simulink model "sf_battery_management"  (R2025b)
settings: Solver=FixedStepAuto  StartTime=0.0  StopTime=inf  FixedStep=0.1  RelTol=1e-3
PreLoadFcn:
  | load('battery_management_data.mat')
values from neighbouring files (symbols this model uses):
  CODEGEN_FLAG = 0    [battery_management_data.mat]
  currentFaultSim = 0    [battery_management_data.mat]
  currentSensorSim = 0    [battery_management_data.mat]
  tempFaultSim = 0    [battery_management_data.mat]
  tempSensorSim = 0    [battery_management_data.mat]
  voltageFaultSim = 0    [battery_management_data.mat]
  voltageSensorSim = 0    [battery_management_data.mat]
(part 3 of 3)

== stateflow chart sf_battery_management/Sensor Readings with Fault Detection ==
  state VoltageSensor [parallel]
    settings: executionOrder=1
    state SensorFaultDetection
      du: sensorError = isError(voltageRead);
      state Valid
        voltage = voltageRead;
        previousReading = voltage;
      state FaultDetected
        voltage = previousReading;
        sensorFaultDetected = true;
      state StandBy
        voltage = previousReading;
      (default) -> VoltageSensor.SensorFaultDetection.Valid
      (junction 159) -> VoltageSensor.SensorFaultDetection.Valid
      VoltageSensor.SensorFaultDetection.FaultDetected -> (junction 159) : [duration(~sensorError) > TIMEOUT]
          | {sensorFaultDetected = false;}
      VoltageSensor.SensorFaultDetection.StandBy -> VoltageSensor.SensorFaultDetection.Valid [order 1] : [~sensorError]
      VoltageSensor.SensorFaultDetection.Valid -> VoltageSensor.SensorFaultDetection.StandBy : [sensorError]
      VoltageSensor.SensorFaultDetection.StandBy -> VoltageSensor.SensorFaultDetection.FaultDetected [order 2] : [duration(sensorError) > TIMEOUT]
    VoltageSensor -> (junction 27)
    (junction 27) -> (junction 29) [order 1] : [CODEGEN_FLAG]
    (junction 27) -> (junction 94) [order 2] : %Sim behavior (dashboard blocks)
    (junction 29) -> (junction 31) : %Codegen behavior (call hardware driver C code)
        | {voltageRead = double(readVoltage())
        | voltageRead = voltageRead / 1000;}
    (junction 94) -> (junction 98) [order 1] : [voltageFaultSim >0]
    (junction 94) -> (junction 71) [order 2] : {voltageRead = voltageSensorSim;
        | voltageRead = voltageRead+VOLTAGE_NOISE*rand();}
    (junction 98) -> (junction 99) : {voltageRead = ERROR;}
    (junction 71) -> (junction 99)
    (junction 99) -> (junction 31)
  state CurrentSensor [parallel]
    settings: executionOrder=2
    state SensorFaultDetection
      du: sensorError = isError(currentRead);
      state Valid
        current = currentRead;
        previousReading = current;
      state FaultDetected
        current = previousReading;
        sensorFaultDetected = true;
      state StandBy
        current = previousReading;
      (default) -> CurrentSensor.SensorFaultDetection.Valid
      (junction 215) -> CurrentSensor.SensorFaultDetection.Valid
      CurrentSensor.SensorFaultDetection.FaultDetected -> (junction 215) : [duration(~sensorError) > TIMEOUT]
          | {sensorFaultDetected = false;}
      CurrentSensor.SensorFaultDetection.StandBy -> CurrentSensor.SensorFaultDetection.Valid [order 1] : [~sensorError]
      CurrentSensor.SensorFaultDetection.Valid -> CurrentSensor.SensorFaultDetection.StandBy : [sensorError]
      CurrentSensor.SensorFaultDetection.StandBy -> CurrentSensor.SensorFaultDetection.FaultDetected [order 2] : [duration(sensorError) > TIMEOUT]
    CurrentSensor -> (junction 111)
    (junction 111) -> (junction 110) [order 1] : [CODEGEN_FLAG]
    (junction 111) -> (junction 115) [order 2] : %Sim behavior (dashboard blocks)
    (junction 110) -> (junction 112) : %Codegen  behavior (call hardware driver C code)
        | {currentRead = double(readCurrent());
        |  currentRead = currentRead / 1000;}
    (junction 115) -> (junction 236) [order 1] : [currentFaultSim >0]
    (junction 115) -> (junction 114) [order 2] : {currentRead = currentSensorSim;
        | currentRead = currentRead+CURRENT_NOISE*rand();}
    (junction 236) -> (junction 118) : {currentRead = ERROR;}
    (junction 114) -> (junction 118)
    (junction 118) -> (junction 112)
  state TemperatureSensor [parallel]
    settings: executionOrder=3
    state SensorFaultDetection
      du: sensorError = isError(tempRead);
      state Valid
        temperature = tempRead;
        previousReading = temperature;
      state FaultDetected
        temperature = previousReading;
        sensorFaultDetected = true;
      state StandBy
        temperature = previousReading;
      (default) -> TemperatureSensor.SensorFaultDetection.Valid
      (junction 227) -> TemperatureSensor.SensorFaultDetection.Valid
      TemperatureSensor.SensorFaultDetection.FaultDetected -> (junction 227) : [duration(~sensorError) > TIMEOUT]
          | {sensorFaultDetected = false;}
      TemperatureSensor.SensorFaultDetection.StandBy -> TemperatureSensor.SensorFaultDetection.Valid [order 1] : [~sensorError]
      TemperatureSensor.SensorFaultDetection.Valid -> TemperatureSensor.SensorFaultDetection.StandBy : [sensorError]
      TemperatureSensor.SensorFaultDetection.StandBy -> TemperatureSensor.SensorFaultDetection.FaultDetected [order 2] : [duration(sensorError) > TIMEOUT]
    TemperatureSensor -> (junction 127)
    (junction 127) -> (junction 126) [order 1] : [CODEGEN_FLAG]
    (junction 127) -> (junction 131) [order 2] : %Sim behavior (dashboard blocks)
    (junction 126) -> (junction 128) : %Codegen behavior (call hardware driver C code)
        | {tempRead = double(readTemperature());
        |  tempRead = tempRead / 1000;}
    (junction 131) -> (junction 136) [order 1] : [tempFaultSim >0]
    (junction 131) -> (junction 130) [order 2] : {tempRead = tempSensorSim;
        | tempRead = tempRead+TEMP_NOISE*rand();}
    (junction 136) -> (junction 134) : {tempRead = ERROR;}
    (junction 130) -> (junction 134)
    (junction 134) -> (junction 128)
  state E = isError(reading) [function]
    (default) -> (junction 191)
    (junction 191) -> (junction 194) [order 1] : [reading < ERROR + ERROR_TOL]
    (junction 191) -> (junction 196) [order 2] : {E = false;}
    (junction 194) -> (junction 198) : {E = true;}
    (junction 198) -> (junction 196)
  data: previousReading local size=1 =0; sensorError local =false; previousReading local size=1 =0; sensorError local =false; previousReading local size=1 =0; sensorError local =false; reading function_input double size=1; E function_output; voltage output double size=1; current output double size=1; temperature output double size=1; voltageRead local double size=1 =-9999; currentRead local double size=1 =0; tempRead local double size=1 =0; CODEGEN_FLAG parameter; voltageSensorSim parameter; voltageFaultSim parameter; currentFaultSim parameter; tempFaultSim parameter; ERROR constant double =-9999; currentSensorSim parameter; tempSensorSim parameter; TIMEOUT constant double =1; VOLTAGE_NOISE constant double =5; ERROR_TOL constant double =10; CURRENT_NOISE constant double =0.5; TEMP_NOISE constant double =3; sensorFaultDetected output boolean

== stateflow chart sf_battery_management/Battery Power Limit Control/Current Limit Control Logic ==
  state BatteryOn
    state Charging
      state FastCharge
        dischargeLimit = CHARGE_FAST;
      state SlowCharge
        dischargeLimit = CHARGE_SLOW;
      (default) -> FastCharge
      FastCharge -> SlowCharge : [batteryState == HIGH]
    state Discharging
      state PerformanceMode
        dischargeLimit = DISCHARGE_MAX;
      state BatterySaverMode
        dischargeLimit = DISCHARGE_LIMITED;
      (default) -> PerformanceMode
      BatterySaverMode -> PerformanceMode : [batteryState  ~= LOW]
      PerformanceMode -> BatterySaverMode : [batteryState == LOW]
    (default) -> Discharging
    Discharging -> Charging [order 1] : [isCharging == true]
    Charging -> Discharging [order 1] : [isCharging == false]
  state BatteryOff
    dischargeLimit = DISCHARGE_OFF;
  (default) -> BatteryOn
  BatteryOff -> Discharging [order 2] : [isCharging == false && batteryState ~= MIN]
  Discharging -> BatteryOff [order 2] : [batteryState == MIN]
  Charging -> BatteryOff [order 2] : [batteryState == MAX]
  BatteryOff -> Charging [order 1] : [isCharging == true && batteryState ~= MAX]
  data: isCharging input boolean; dischargeLimit output; DISCHARGE_MAX constant double =2; DISCHARGE_LIMITED constant double =1; DISCHARGE_OFF constant double =0; CHARGE_SLOW constant double =-1; CHARGE_FAST constant double =-2; batteryState input Enum: BatteryStates

== stateflow chart sf_battery_management/Battery State Estimation ==
  state BatteryStateDebouncer
    SOC = estimateSOC(voltage,current,temperature)*100;
    state BatteryMax
      batteryState = MAX;
    state BatteryHigh
      batteryState = HIGH;
    state Normal
      batteryState = NORMAL;
    state BatteryLow
      batteryState = LOW;
    state BatteryMin
      batteryState = MIN;
    (default) -> (junction 39)
    (junction 39) -> BatteryMax [order 1] : [SOC > SOC_MAX]
    BatteryMax -> BatteryStateDebouncer : [duration(SOC < SOC_MAX) > HOLD_TIME]
    (junction 39) -> (junction 40) [order 2]
    (junction 40) -> BatteryHigh [order 1] : [SOC > SOC_HIGH]
    BatteryHigh -> BatteryStateDebouncer : [duration(SOC < SOC_HIGH || ...
        | SOC > SOC_MAX) > HOLD_TIME]
    (junction 40) -> (junction 41) [order 2]
    (junction 41) -> Normal [order 1] : [SOC > SOC_LOW]
    Normal -> BatteryStateDebouncer : [duration(SOC < SOC_LOW || ...
        | SOC > SOC_HIGH) > HOLD_TIME]
    (junction 41) -> (junction 42) [order 2]
    (junction 42) -> BatteryLow [order 1] : [SOC > SOC_MIN]
    BatteryLow -> BatteryStateDebouncer : [duration(SOC < SOC_MIN || ...
        | SOC > SOC_LOW) > HOLD_TIME]
    (junction 42) -> (junction 43) [order 2]
    (junction 43) -> BatteryMin
    BatteryMin -> BatteryStateDebouncer : [duration(SOC > SOC_MIN) > HOLD_TIME]
  data: voltage input; current input; temperature input; batteryState output Enum: BatteryStates; SOC_MIN constant double =15; SOC_MAX constant double =95; SOC_LOW constant double =30; SOC_HIGH constant double =80; HOLD_TIME constant double =3; SOC local double =0
